simulink model "MyHistogramEqualizationForHDLCoder2"  (R2024b)
settings: Solver=VariableStepAuto  StartTime=0.0  StopTime=10.0  RelTol=1e-3
undefined symbols (not defined in the file): gray
libraries: visionsources x1
settings Model: Creator=snmz4  LastModifiedBy=snmz4

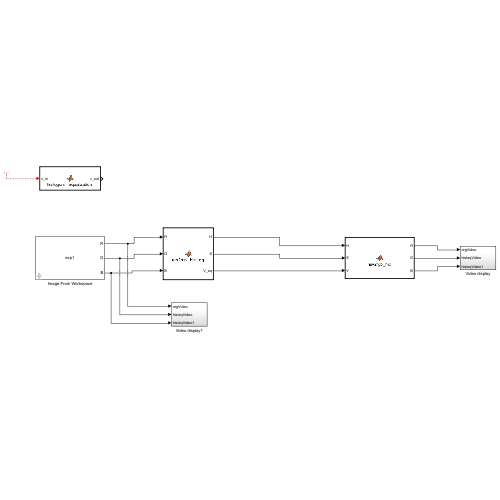
[thumbnail: Simulink's stored preview of the top-level diagram]
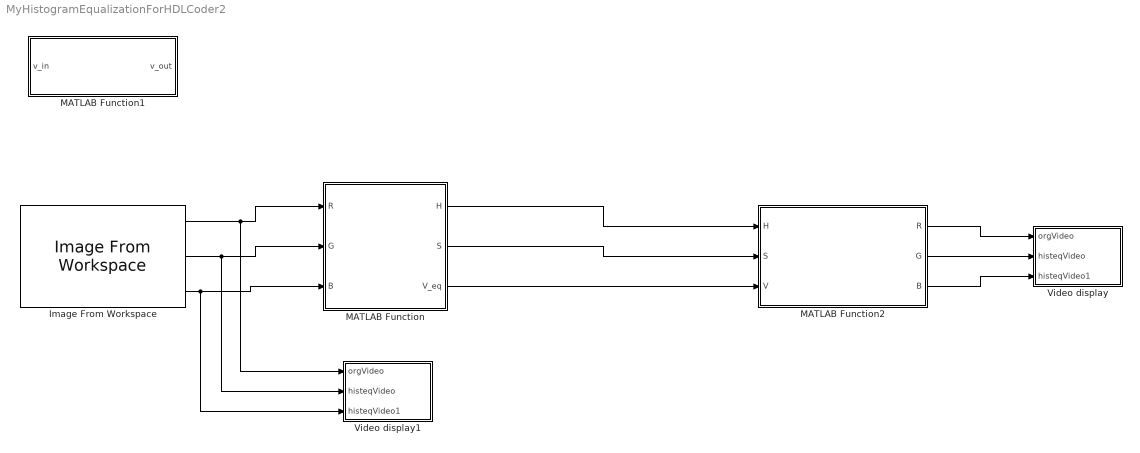
== system MyHistogramEqualizationForHDLCoder2 ==
  Image From Workspace : visionsources/Image From Workspace  Tag=vipblks_nd  ImageValue=exp1  Ts=inf  imagePorts=Separate color signals  OutPortLabels=R|G|B  ImageDataType=uint8  Signed=on  WordLength=16  sdImageDataType=sfix(16)  FractionLengthMode=User-defined  FractionLength=15
  MATLAB Function : MATLAB Function  TreatAsAtomicUnit=on
  MATLAB Function1 : MATLAB Function  TreatAsAtomicUnit=on
  MATLAB Function2 : MATLAB Function  TreatAsAtomicUnit=on
  Video display : Subsystem
  Video display1 : Subsystem
  wires:
  ? -> MATLAB Function1/1(v_in)
  MATLAB Function/1(H) -> MATLAB Function2/1(H)
  MATLAB Function/2(S) -> MATLAB Function2/2(S)
  MATLAB Function2/1(R) -> Video display/1(orgVideo)
  MATLAB Function2/2(G) -> Video display/2(histeqVideo)
  MATLAB Function2/3(B) -> Video display/3(histeqVideo1)
  MATLAB Function/3(V_eq) -> MATLAB Function2/3(V)
  Image From Workspace/2 -> Video display1/2(histeqVideo), MATLAB Function/2(G)
  Image From Workspace/3 -> Video display1/3(histeqVideo1), MATLAB Function/3(B)
  Image From Workspace/1 -> Video display1/1(orgVideo), MATLAB Function/1(R)

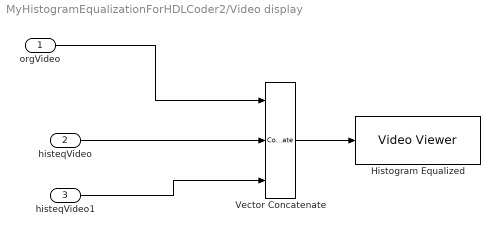
== system MyHistogramEqualizationForHDLCoder2/Video display ==
  orgVideo : Inport
  histeqVideo : Inport  Port=2
  histeqVideo1 : Inport  Port=3
  Histogram Equalized : VideoViewer  colormapValue=gray(256)  specRange=on  FigPos=[663.4 658.8 765.6 431.2]  trueSizedOnce=on
  Vector Concatenate : Concatenate  NumInputs=3  Mode=Multidimensional array  ConcatenateDimension=3
  wires:
  histeqVideo/1 -> Vector Concatenate/2
  orgVideo/1 -> Vector Concatenate/1
  Vector Concatenate/1 -> Histogram Equalized/1
  histeqVideo1/1 -> Vector Concatenate/3

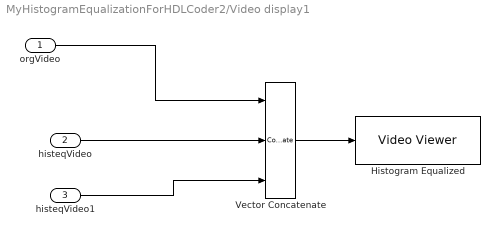
== system MyHistogramEqualizationForHDLCoder2/Video display1 ==
  orgVideo : Inport
  histeqVideo : Inport  Port=2
  histeqVideo1 : Inport  Port=3
  Histogram Equalized : VideoViewer  colormapValue=gray(256)  specRange=on  FigPos=[44.2 661.2 765.6 431.2]  trueSizedOnce=on
  Vector Concatenate : Concatenate  NumInputs=3  Mode=Multidimensional array  ConcatenateDimension=3
  wires:
  histeqVideo/1 -> Vector Concatenate/2
  orgVideo/1 -> Vector Concatenate/1
  Vector Concatenate/1 -> Histogram Equalized/1
  histeqVideo1/1 -> Vector Concatenate/3

== matlab function MyHistogramEqualizationForHDLCoder2/MATLAB Function1 ==
  data: v_in input; v_out output
function v_out = histogram_equalization(v_in)
%#codegen

persistent hist cdf

% Çıkış boyutunu ve türünü belirleme
v_out = coder.nullcopy(zeros(size(v_in), 'uint8')); 

if isempty(hist)
    hist = fi(zeros(1,256), 0, 16, 0); % 16-bit sabit nokta histogram
    cdf  = fi(zeros(1,256), 0, 16, 0); % 16-bit sabit nokta CDF
end

% Histogram hesaplama
for i = 1:length(v_in)
    hist(v_in(i) + 1) = hist(v_in(i) + 1) + 1;
end

% Kümülatif dağılım fonksiyonu (CDF) hesaplama
cdf(1) = hist(1);
for j = 2:256
    cdf(j) = cdf(j-1) + hist(j); 
end

% Normalize etme (CDF'nin son elemanına göre normalize et)
max_cdf_value = double(cdf(256)); % veya cdf(end)
% Normalize edilmiş CDF'yi farklı bir değişkende saklayın
cdf_norm = fi(255 * double(cdf) / max_cdf_value, 0, 16, 0); 

% Yeni parlaklık değerlerini eşitleme
for i = 1:length(v_in)
    v_out(i) = uint8(double(cdf_norm(v_in(i) + 1))); 
end

end

== matlab function MyHistogramEqualizationForHDLCoder2/MATLAB Function ==
  data: R input; H output; S output; V_eq output; G input; B input
function [H, S, V_eq] = rgb2hsv_hist_eq(R, G, B)
%#codegen
% Bu fonksiyon, girişteki R, G, B kanallarını kullanarak RGB -> HSV
% dönüşümü gerçekleştirir. Ardından hesaplanan Value (V) kanalına 
% histogram equalization uygular.
%
% Girişler:
%   R, G, B - [270x372] uint8 matrisler. (Her biri 0-255 aralığında değer içerir)
%
% Çıkışlar:
%   H    - [270x372] double matris, hue değeri (0 ile 360 derece arasında)
%   S    - [270x372] double matris, saturation (0 ile 1 aralığında)
%   V_eq - [270x372] double matris, histogram equalize edilmiş value (0 ile 1 aralığında)

% Sabit boyutlar
rows = 270;
cols = 372;

%% 1. AŞAMA: RGB -> HSV DÖNÜŞÜMÜ
H = zeros(rows, cols);
S = zeros(rows, cols);
V = zeros(rows, cols);

for i = 1:rows
    for j = 1:cols
        % RGB değerlerini normalize et (0-255'ten 0-1'e)
        r_val = double(R(i, j)) / 255;
        g_val = double(G(i, j)) / 255;
        b_val = double(B(i, j)) / 255;
        
        % Maksimum ve minimum değeri belirle
        max_val = r_val;
        if g_val > max_val
            max_val = g_val;
        end
        if b_val > max_val
            max_val = b_val;
        end
        
        min_val = r_val;
        if g_val < min_val
            min_val = g_val;
        end
        if b_val < min_val
            min_val = b_val;
        end
        
        delta = max_val - min_val;
        
        % Hesaplanan Value değeri
        V(i, j) = max_val;
        
        % Saturation hesaplaması
        if max_val == 0  
            S(i, j) = 0;
        else
            S(i, j) = delta / max_val;
        end
        
        % Hue hesaplaması
        if delta == 0
            H(i, j) = 0;
        else
            if r_val == max_val
                h_val = (g_val - b_val) / delta;
            elseif g_val == max_val
                h_val = 2 + (b_val - r_val) / delta;
            else  % b_val == max_val
                h_val = 4 + (r_val - g_val) / delta;
            end
            
            h_val = h_val * 60;  % Dereceye çevirme
            if h_val < 0
                h_val = h_val + 360;
            end
            H(i, j) = h_val;
        end
    end
end

%% 2. AŞAMA: Histogram Equalization - Value (V) Kanalı
% Histogram equalization için standart 256 seviye kullanıyoruz.
levels = 256;
totalPixels = rows * cols;

% Adım 2.1: V kanalındaki değerleri [0, levels-1] aralığına ölçeklendir.
V_int = zeros(rows, cols, 'uint8');
for i = 1:rows
    for j = 1:cols
        % V değeri [0,1] aralığında olduğundan, *255 işlemi ile 0-255 aralığına
        % dönüşüm yapılır; burada yuvarlama işlemi floor ile yapılıyor.
        V_int(i,j) = uint8(floor(V(i, j)*(levels-1) + 0.5));
    end
end

% Adım 2.2: Histogram hesaplama (256 adet seviye için)
histogram = zeros(levels,1);
for i = 1:rows
    for j = 1:cols
         bin = double(V_int(i,j));  % 0'dan 255'e kadar
         % MATLAB dizinleme 1'den başladığı için: bin+1
         histogram(bin+1) = histogram(bin+1) + 1;
    end
end

% Adım 2.3: Kümülatif dağılım fonksiyonunu (CDF) hesapla.
cdf = zeros(levels,1);
cdf(1) = histogram(1);
for k = 2:levels
    cdf(k) = cdf(k-1) + histogram(k);
end

% Adım 2.4: cdf_min değerini belirle (ilk sıfırdan farklı değeri)
cdf_min = 0;
for k = 1:levels
    if cdf(k) > 0
        cdf_min = cdf(k);
        break;
    end
end

% Adım 2.5: Eşitleme dönüşümünü uygula.
V_eq = zeros(rows, cols);
for i = 1:rows
    for j = 1:cols
         bin = double(V_int(i,j));
         % Yeni pixel değeri hesaplanıyor (0-1 aralığında)
         V_eq(i,j) = (cdf(bin+1) - cdf_min) / (totalPixels - cdf_min);
    end
end

end

== matlab function MyHistogramEqualizationForHDLCoder2/MATLAB Function2 ==
  data: H input; R output; S input; V input; G output; B output
function [R, G, B] = hsv2rgb_hdl(H, S, V)
%#codegen
% Bu fonksiyon, histogram equalization uygulanmış V değeriyle birlikte
% H ve S kanallarından RGB dönüşümü gerçekleştirir.
%
% Girişler:
%   H - [270x372] double matris, hue değeri (0 ile 360 derece arası)
%   S - [270x372] double matris, saturation (0 ile 1 arasında)
%   V - [270x372] double matris, histogram equalization uygulanmış value (0 ile 1 arasında)
%
% Çıkışlar:
%   R, G, B - [270x372] uint8 matrisler, 0-255 aralığında RGB değerleri

% Sabit boyutlar
rows = 270;
cols = 372;

% Çıkış dizilerini önceden tanımla.
R = zeros(rows, cols, 'uint8');
G = zeros(rows, cols, 'uint8');
B = zeros(rows, cols, 'uint8');

for i = 1:rows
    for j = 1:cols
        % Her bir piksel için HSV değerlerini oku.
        h = H(i, j);
        s = S(i, j);
        v = V(i, j);
        
        % Güvenlik: Eğer h 360 veya daha büyükse hue 0 kabul edilir.
        if h >= 360
            h = 0;
        end
        
        % Eğer doyma yoksa renk gri tonlardadır.
        if s == 0
            r_val = v;
            g_val = v;
            b_val = v;
        else
            % HSV -> RGB dönüşümü:
            % Hue değeri 60'a bölünerek hangi segmentte olduğumuz bulunur.
            h_sector = h / 60.0;
            i_sector = floor(h_sector);  % Bu değer 0 ile 5 arasında olacaktır.
            f = h_sector - i_sector;
            
            % Ara değerler hesaplanıyor.
            p = v * (1 - s);
            q = v * (1 - s * f);
            t = v * (1 - s * (1 - f));
            
            % i_sector değerine göre RGB hesaplanıyor.
            if i_sector == 0
                r_val = v;
                g_val = t;
                b_val = p;
            elseif i_sector == 1
                r_val = q;
                g_val = v;
                b_val = p;
            elseif i_sector == 2
                r_val = p;
                g_val = v;
                b_val = t;
            elseif i_sector == 3
                r_val = p;
                g_val = q;
                b_val = v;
            elseif i_sector == 4
                r_val = t;
                g_val = p;
                b_val = v;
            elseif i_sector == 5
                r_val = v;
                g_val = p;
                b_val = q;
            else
                % Bu durum normalde gerçekleşmez; güvenlik için.
                r_val = v;
                g_val = v;
                b_val = v;
            end
        end
        
        % 0-1 aralığındaki değerleri 0-255 aralığına ölçeklendirip uint8 çeviriyoruz.
        R(i, j) = uint8(r_val * 255);
        G(i, j) = uint8(g_val * 255);
        B(i, j) = uint8(b_val * 255);
    end
end

end
